simulink model "sm_car"  (R2025a)
settings: Solver=ode23t  StartTime=0.0  StopTime=400  MaxStep=0.4  RelTol=1e-3  AbsTol=1e-3  EnableMultiTasking=on
PreLoadFcn:
  | % Due to usability issue in Repeating Sequence block
  | warning('off','Simulink:Masking:Invalid');
  | 
  | % Eliminate unnecessary warnings in inactive variants
  | % Warnings generated only if you click through inactive variant
  | warning('off','MATLAB:nonExistentField');
  | warning('off','Simulink:Parameters:BlkParamUndefined');
PostLoadFcn:
  | set_param([bdroot '/Vehicle'],'popup_trailer','Off')
  | warning('off','sm:sli:setup:compile:LocalSolverNotSupported')
  | %sm_car_config_maneuver(bdroot,'WOT Braking');
  | sm_car_config_vehicle(bdroot,'false');
  | sm_car_config_logging(bdroot);
InitFcn:
  | sm_car_config_camera;
  | Vehicle = sm_car_vehcfg_checkConfig(Vehicle);
  | sm_car_check_tire_model(bdroot);
StartFcn:
  | tic;
StopFcn:
  | Elapsed_Sim_Time = toc;
  | % disp(['Elapsed Sim Time = ' num2str(Elapsed_Sim_Time)]);
undefined symbols (not defined in the file): Axle1D, AxleIn, Camera, Control, Driver, Free, Init, Maneuver, Pedal, RaceFix, RaceSpin, Scene, ShaftL1, ShaftL2, ShaftR1, ShaftR2, Soft, Stiff, Visual, X, xy_data_car_side, Y, Z
libraries: sm_lib x1546, nesl_utility x528, fl_lib x480, SimscapeFluids_lib x61, sdl_lib x49, simulink x29, ee_lib x7, simulink_extras x6, Linkage_Systems x4, Tire_1x2x x4, AntiRollBar_Systems x2, Linkage_Decoupled x2
(part 9 of 79)

== system sm_car/World/Scene/Skidpad/Circle Outer R ==
  Solid : sm_lib/Body Elements/Extruded Solid  ExtrusionType=General  PolygonNumSides=3  PolygonOuterRadius=1  PolygonOuterRadiusUnits=m  ExportEntireGeometry=off  ExtrusionCrossSection=xy_data_circ  ExtrusionCrossSectionUnits=m  ExportConvexHullGeometry=off  ExtrusionLength=circ_h  ExtrusionLengthUnits=m  InertiaType=CalculateFromGeometry  BasedOnType=Density  Density=1000  DensityUnits=kg/m^3  Mass=1  MassUnits=kg  CenterOfMass=[0 0 0]  CenterOfMassUnits=m  MomentsOfInertia=[1 1 1]  MomentsOfInertiaUnits=kg*m^2  ProductsOfInertia=[1 1 1]  ProductsOfInertiaUnits=kg*m^2  GraphicType=FromGeometry  MarkerShape=Sphere  MarkerSize=10  GraphicVisPropType=SimpleVisualProperties  GraphicDiffuseColor=[1.0 1.0 0.8]  GraphicOpacity=1.0  GraphicSpecularColor=[0.5 0.5 0.5 1.0]  GraphicAmbientColor=[0.15 0.15 0.15 1.0]  GraphicEmissiveColor=[0.0 0.0 0.0 1.0]  GraphicShininess=75  DoExposeReferenceFrame=on  SerializedFrames=<Frames/>
  W : PMIOPort  Side=Right
  connections:
  Solid/RConn1 -- W/RConn1

== system sm_car/World/Scene/Skidpad/Ground Plane ==
  Floor : sm_lib/Body Elements/Brick Solid  BrickDimensions=[gp_l, gp_w, gp_h]  BrickDimensionsUnits=m  ExportEntireGeometry=off  InertiaType=CalculateFromGeometry  BasedOnType=Density  Density=1000  DensityUnits=kg/m^3  Mass=1  MassUnits=kg  CenterOfMass=[0 0 0]  CenterOfMassUnits=m  MomentsOfInertia=[1 1 1]  MomentsOfInertiaUnits=kg*m^2  ProductsOfInertia=[0 0 0]  ProductsOfInertiaUnits=kg*m^2  GraphicType=FromGeometry  MarkerShape=Sphere  MarkerSize=10  GraphicVisPropType=SimpleVisualProperties  GraphicDiffuseColor=gp_clr  GraphicOpacity=gp_opc  GraphicSpecularColor=[0.5 0.5 0.5 1.0]  GraphicAmbientColor=[0.15 0.15 0.15 1.0]  GraphicEmissiveColor=[0.0 0.0 0.0 1.0]  GraphicShininess=75  DoExposeReferenceFrame=off  SerializedFrames=<Frames><Frame><Id>Frame1</Id><Value><Name>F</Name><Origin><Source>GeometricFeature</Source><FeatureName>+z surface</FeatureName></Origin><PrimaryAxis><DefinedDirection>+Z</DefinedDirection><Source>ReferenceFrame</Source><SourceDirection>+Z</SourceDirection><FeatureName></FeatureName></PrimaryAxis><SecondaryAxis><DefinedDirection>+X</DefinedDirection><Source>ReferenceFrame</Source><SourceDirection>+X</SourceDirection><FeatureName></FeatureName></SecondaryAxis></Value></Frame></Frames>
  W : PMIOPort  Side=Right
  connections:
  Floor/LConn1 -- W/RConn1

== system sm_car/Controller/Default/Damper Control/Damper Control A1/None ==
  mL : Inport
  mR : Inport  Port=2
  Inp : Inport  Port=3
  Ground : Ground
  Ground1 : Ground
  Terminator : Terminator
  Terminator1 : Terminator
  Terminator2 : Terminator
  L : Outport  VectorParamsAs1DForOutWhenUnconnected=off
  R : Outport  Port=2  VectorParamsAs1DForOutWhenUnconnected=off
  wires:
  Inp/1 -> Terminator2/1
  mR/1 -> Terminator1/1
  mL/1 -> Terminator/1
  Ground1/1 -> R/1  "R"
  Ground/1 -> L/1  "L"

== system sm_car/Controller/Default/Damper Control/Damper Control A2/None ==
  mL : Inport
  mR : Inport  Port=2
  Inp : Inport  Port=3
  Ground : Ground
  Ground1 : Ground
  Terminator : Terminator
  Terminator1 : Terminator
  Terminator2 : Terminator
  L : Outport  VectorParamsAs1DForOutWhenUnconnected=off
  R : Outport  Port=2  VectorParamsAs1DForOutWhenUnconnected=off
  wires:
  Inp/1 -> Terminator2/1
  mR/1 -> Terminator1/1
  mL/1 -> Terminator/1
  Ground1/1 -> R/1  "R"
  Ground/1 -> L/1  "L"

== system sm_car/Controller/Default/Spring Control/Spring Control A1/Hydropneumatic ==
  mL : Inport
  mR : Inport  Port=2
  Inp : Inport  Port=3
  Bus Creator : BusCreator  Inputs=5
  Constant : Constant  Value=0
  Constant1 : Constant  Value=0
  Gain : Gain
  Prop Damper : Constant  Value=0
  Soft Suspension : Constant  Value=soft_suspension
  Terminator : Terminator
  Terminator1 : Terminator
  Terminator2 : Terminator
  L : Outport  VectorParamsAs1DForOutWhenUnconnected=off
  R : Outport  Port=2  VectorParamsAs1DForOutWhenUnconnected=off
  wires:
  Bus Creator/1 -> R/1, L/1  "R"
  mL/1 -> Terminator/1
  mR/1 -> Terminator1/1
  Inp/1 -> Terminator2/1
  Constant1/1 -> Bus Creator/5  "RideHeightOut"
  Gain/1 -> Bus Creator/1  "GasSprStiff"
  Soft Suspension/1 -> Bus Creator/2, Gain/1  "GasSprSoft"
  Prop Damper/1 -> Bus Creator/3  "Damper"
  Constant/1 -> Bus Creator/4  "RideHeightIn"

== system sm_car/Controller/Default/Spring Control/Spring Control A1/None ==
  mL : Inport
  mR : Inport  Port=2
  Inp : Inport  Port=3
  Ground : Ground
  Ground1 : Ground
  Terminator1 : Terminator
  Terminator2 : Terminator
  Terminator3 : Terminator
  L : Outport  VectorParamsAs1DForOutWhenUnconnected=off
  R : Outport  Port=2  VectorParamsAs1DForOutWhenUnconnected=off
  wires:
  Inp/1 -> Terminator3/1
  Ground/1 -> L/1  "L"
  Ground1/1 -> R/1  "R"
  mL/1 -> Terminator1/1
  mR/1 -> Terminator2/1

== system sm_car/Controller/Default/Spring Control/Spring Control A2/Hydropneumatic ==
  mL : Inport
  mR : Inport  Port=2
  Inp : Inport  Port=3
  Bus Creator : BusCreator  Inputs=5
  Constant : Constant  Value=0
  Constant1 : Constant  Value=0
  Gain : Gain
  Prop Damper : Constant  Value=0
  Soft Suspension : Constant  Value=soft_suspension
  Terminator : Terminator
  Terminator1 : Terminator
  Terminator2 : Terminator
  L : Outport  VectorParamsAs1DForOutWhenUnconnected=off
  R : Outport  Port=2  VectorParamsAs1DForOutWhenUnconnected=off
  wires:
  Bus Creator/1 -> R/1, L/1  "R"
  mL/1 -> Terminator/1
  mR/1 -> Terminator1/1
  Inp/1 -> Terminator2/1
  Constant1/1 -> Bus Creator/5  "RideHeightOut"
  Gain/1 -> Bus Creator/1  "GasSprStiff"
  Soft Suspension/1 -> Bus Creator/2, Gain/1  "GasSprSoft"
  Prop Damper/1 -> Bus Creator/3  "Damper"
  Constant/1 -> Bus Creator/4  "RideHeightIn"

== system sm_car/Controller/Default/Spring Control/Spring Control A2/None ==
  mL : Inport
  mR : Inport  Port=2
  Inp : Inport  Port=3
  Ground : Ground
  Ground1 : Ground
  Terminator1 : Terminator
  Terminator2 : Terminator
  Terminator3 : Terminator
  L : Outport  VectorParamsAs1DForOutWhenUnconnected=off
  R : Outport  Port=2  VectorParamsAs1DForOutWhenUnconnected=off
  wires:
  Inp/1 -> Terminator3/1
  Ground/1 -> L/1  "L"
  Ground1/1 -> R/1  "R"
  mL/1 -> Terminator1/1
  mR/1 -> Terminator2/1

== system sm_car/Controller/TrqVec 4Motor/Brake Control/ABS/Calculate Slip ==
  WhlSpd : Inport
  VehSpdEst : Inport  Port=2
  Abs : Abs  ZeroCross=off  SaturateOnIntegerOverflow=off
  Bus Creator : BusCreator  Inputs=4
  Bus Selector1 : BusSelector  OutputSignals=L1.v,R1.v,L2.v,R2.v
  Constant : Constant
  Demux : Demux
  Fcn{,1..3} (4 alike) : Fcn  Expr=abs(u(1)*u(2)-u(3))/u(3)
  Mux{,1..3} (4 alike) : Mux  Inputs=3
  Mux4 : Mux
  Mux5 : Mux
  Product : Product
  Saturation : Saturate  UpperLimit=inf  LowerLimit=eps  ZeroCross=off
  Saturation1 : Saturate  UpperLimit=1  LowerLimit=0
  Sign : Signum  ZeroCross=off
  Wheel Speeds and Slip : Scope  NumInputPorts=2
      settings: ActiveDisplayYMinimum=-11.64241  ActiveDisplayYMaximum=114.01232  DataLoggingVariableName=ScopeData2
  Slip : Outport  VectorParamsAs1DForOutWhenUnconnected=off
  wires:
  WhlSpd/1 -> Bus Selector1/1
  Bus Selector1/2 -> Mux4/2, Mux1/2  "<v>"
  Bus Selector1/4 -> Mux4/4, Mux3/2  "<v>"
  Bus Selector1/1 -> Mux4/1, Mux/2  "<v>"
  Bus Selector1/3 -> Mux4/3, Mux2/2  "<v>"
  Constant/1 -> Mux/1, Mux1/1, Mux3/1, Mux2/1
  VehSpdEst/1 -> Sign/1, Abs/1
  Demux/1 -> Bus Creator/1  "L1"
  Demux/2 -> Bus Creator/2  "R1"
  Demux/3 -> Bus Creator/3  "L2"
  Demux/4 -> Bus Creator/4  "R2"
  Bus Creator/1 -> Wheel Speeds and Slip/2, Slip/1  "Slip"
  Product/1 -> Mux3/3, Mux2/3, Mux1/3, Mux/3
  Abs/1 -> Saturation/1
  Saturation/1 -> Product/1
  Sign/1 -> Product/2
  Mux/1 -> Fcn/1
  Mux1/1 -> Fcn1/1
  Mux2/1 -> Fcn2/1
  Mux3/1 -> Fcn3/1
  Mux4/1 -> Wheel Speeds and Slip/1  "Wheel Speeds"
  Mux5/1 -> Saturation1/1
  Saturation1/1 -> Demux/1
  Fcn/1 -> Mux5/1  "L1"
  Fcn1/1 -> Mux5/2  "R1"
  Fcn2/1 -> Mux5/3  "L2"
  Fcn3/1 -> Mux5/4  "R2"

== system sm_car/Controller/TrqVec 4Motor/Brake Control/ABS/Sensor ==
  Body : Inport
  WhlSpd : Inport  Port=2
  Bus Creator{,3..5} (4 alike) : BusCreator  Inputs=1
  Bus Creator6 : BusCreator  Inputs=5
  Bus Selector : BusSelector  OutputSignals=vx,vy  OutputAsBus=on
  Bus Selector4 : BusSelector  OutputSignals=WhlL1.n,WhlR1.n,WhlL2.n,WhlR2.n,WhlL2.qxyz
  Gain : Gain  Gain=3.6*abs_tire_radiusF
  Gain1 : Gain  Gain=3.6*abs_tire_radiusF
  Gain2 : Gain  Gain=3.6*abs_tire_radiusR
  Gain3 : Gain  Gain=3.6*abs_tire_radiusR
  Gain4 : Gain  Gain=3.6
  Terminator1 : Terminator  Commented=on
  Vel in xy plane : Fcn  Expr=sqrt(u(1)^2+u(2)^2)
  missing tooth : Subsystem  Commented=on
  GroundSpd : Outport  VectorParamsAs1DForOutWhenUnconnected=off
  wires:
  Gain1/1 -> Bus Creator3/1  "v"
  missing tooth/1(Out1) -> Terminator1/1  "v"
  Gain2/1 -> Bus Creator4/1  "v"
  Bus Selector4/5 -> missing tooth/2(<qxyz>)  "<qxyz>"
  Bus Creator5/1 -> Bus Creator6/5  "R2"
  Gain3/1 -> Bus Creator5/1  "v"
  Bus Creator/1 -> Bus Creator6/2  "L1"
  Bus Selector4/2 -> Gain1/1  "<n>"
  Bus Creator4/1 -> Bus Creator6/4  "L2"
  Bus Selector4/3 -> Gain2/1, missing tooth/1(<omega>)  "<n>"
  Gain/1 -> Bus Creator/1  "v"
  Body/1 -> Bus Selector/1
  Bus Creator3/1 -> Bus Creator6/3  "R1"
  Gain4/1 -> Bus Creator6/1  "v"
  Bus Selector4/1 -> Gain/1  "<n>"
  Bus Selector4/4 -> Gain3/1  "<n>"
  WhlSpd/1 -> Bus Selector4/1
  Bus Creator6/1 -> GroundSpd/1
  Vel in xy plane/1 -> Gain4/1  "speed"
  Bus Selector/1 -> Vel in xy plane/1

== system sm_car/Controller/TrqVec 4Motor/Brake Control/ABS/Valve Control L1 ==
  Slip : Inport
  vSpdEst : Inport  Port=2
  Categorize Surface : Subsystem
  Code to Valves : Subsystem
  Demux : Demux  Outputs=2
  Logic : Stateflow chart  TreatAsAtomicUnit=on
  Mux : Mux  Inputs=2
  Product : Product
  Subsystem : Subsystem
  Subsystem1 : Subsystem
  Valve : Outport  VectorParamsAs1DForOutWhenUnconnected=off
  wires:
  Logic/1(Mod_State) -> Categorize Surface/1(Mod State), Code to Valves/1(C)
  Logic/2(Mod_Dur) -> Product/2
  Slip/1 -> Logic/1(Slip)
  Code to Valves/1(V) -> Product/1
  vSpdEst/1 -> Logic/2(vSpdEst)
  Product/1 -> Demux/1
  Demux/1 -> Subsystem/1(OnT)
  Demux/2 -> Subsystem1/1(OnT)
  Mux/1 -> Valve/1
  Subsystem/1(vSig) -> Mux/1, Categorize Surface/2(Apply Valve)
  Subsystem1/1(vSig) -> Mux/2

== system sm_car/Controller/TrqVec 4Motor/Brake Control/ABS/Valve Control L2 ==
  Slip : Inport
  vSpdEst : Inport  Port=2
  Categorize Surface : Subsystem
  Code to Valves : Subsystem
  Demux : Demux  Outputs=2
  Logic : Stateflow chart  TreatAsAtomicUnit=on
  Mux : Mux  Inputs=2
  Product : Product
  Subsystem : Subsystem
  Subsystem1 : Subsystem
  Valve : Outport  VectorParamsAs1DForOutWhenUnconnected=off
  wires:
  Logic/1(Mod_State) -> Categorize Surface/1(Mod State), Code to Valves/1(C)
  Logic/2(Mod_Dur) -> Product/2
  Slip/1 -> Logic/1(Slip)
  Code to Valves/1(V) -> Product/1
  vSpdEst/1 -> Logic/2(vSpdEst)
  Product/1 -> Demux/1
  Demux/1 -> Subsystem/1(OnT)
  Demux/2 -> Subsystem1/1(OnT)
  Mux/1 -> Valve/1
  Subsystem/1(vSig) -> Mux/1, Categorize Surface/2(Apply Valve)
  Subsystem1/1(vSig) -> Mux/2

== system sm_car/Controller/TrqVec 4Motor/Brake Control/ABS/Valve Control R1 ==
  Slip : Inport
  vSpdEst : Inport  Port=2
  Categorize Surface : Subsystem
  Code to Valves : Subsystem
  Demux : Demux  Outputs=2
  Logic : Stateflow chart  TreatAsAtomicUnit=on
  Mux : Mux  Inputs=2
  Product : Product
  Subsystem : Subsystem
  Subsystem1 : Subsystem
  Valve : Outport  VectorParamsAs1DForOutWhenUnconnected=off
  wires:
  Logic/1(Mod_State) -> Categorize Surface/1(Mod State), Code to Valves/1(C)
  Logic/2(Mod_Dur) -> Product/2
  Slip/1 -> Logic/1(Slip)
  Code to Valves/1(V) -> Product/1
  vSpdEst/1 -> Logic/2(vSpdEst)
  Product/1 -> Demux/1
  Demux/1 -> Subsystem/1(OnT)
  Demux/2 -> Subsystem1/1(OnT)
  Mux/1 -> Valve/1
  Subsystem/1(vSig) -> Mux/1, Categorize Surface/2(Apply Valve)
  Subsystem1/1(vSig) -> Mux/2

== system sm_car/Controller/TrqVec 4Motor/Brake Control/ABS/Valve Control R2 ==
  Slip : Inport
  vSpdEst : Inport  Port=2
  Categorize Surface : Subsystem
  Code to Valves : Subsystem
  Demux : Demux  Outputs=2
  Logic : Stateflow chart  TreatAsAtomicUnit=on
  Mux : Mux  Inputs=2
  Product : Product
  Subsystem : Subsystem
  Subsystem1 : Subsystem
  Valve : Outport  VectorParamsAs1DForOutWhenUnconnected=off
  wires:
  Logic/1(Mod_State) -> Categorize Surface/1(Mod State), Code to Valves/1(C)
  Logic/2(Mod_Dur) -> Product/2
  Slip/1 -> Logic/1(Slip)
  Code to Valves/1(V) -> Product/1
  vSpdEst/1 -> Logic/2(vSpdEst)
  Product/1 -> Demux/1
  Demux/1 -> Subsystem/1(OnT)
  Demux/2 -> Subsystem1/1(OnT)
  Mux/1 -> Valve/1
  Subsystem/1(vSig) -> Mux/1, Categorize Surface/2(Apply Valve)
  Subsystem1/1(vSig) -> Mux/2

== system sm_car/Controller/TrqVec 4Motor/Brake Control/ABS/Vehicle Speed ==
  Sensors : Inport
  Bus Selector : BusSelector  OutputSignals=v
  vSpdEst : Outport  VectorParamsAs1DForOutWhenUnconnected=off
  wires:
  Sensors/1 -> Bus Selector/1
  Bus Selector/1 -> vSpdEst/1  "<v>"

== system sm_car/Controller/TrqVec 4Motor/Damper Control/Damper Control A1/Coefficient ==
  mL : Inport
  mR : Inport  Port=2
  Inp : Inport  Port=3
  Bus Selector : BusSelector  OutputSignals=vDamper
  Bus Selector1 : BusSelector  OutputSignals=vDamper
  Demux : Demux  Outputs=2
  Filter : Subsystem  mask(First-order lag supporting vector signals){b=b_A1, x_initial=[0 0]}
      mask prompts: b "Filter time constant"; x_initial "Initial output"
      mask help: Models a lag of the form 1/(b*s+1) where s is the Laplace operator.
  Lookup Table Coeff : Lookup_n-D  BreakpointsForDimension1=brkPts_dim1_A1  BreakpointsForDimension2=brkPts_dim2_A1  Table=Table_A1  InternalRulePriority=Speed  RndMeth=Simplest
      settings: InputPortMap=u0,u1
  Mux1 : Mux  Inputs=2
  L : Outport  VectorParamsAs1DForOutWhenUnconnected=off
  R : Outport  Port=2  VectorParamsAs1DForOutWhenUnconnected=off
  wires:
  Bus Selector1/1 -> Mux1/2  "<vDamper>"
  mR/1 -> Bus Selector1/1
  mL/1 -> Bus Selector/1
  Filter/1(Out) -> Lookup Table Coeff/1  "vDamper"
  Bus Selector/1 -> Mux1/1  "<vDamper>"
  Mux1/1 -> Filter/1(In)
  Demux/1 -> L/1  "L"
  Demux/2 -> R/1  "R"
  Inp/1 -> Lookup Table Coeff/2
  Lookup Table Coeff/1 -> Demux/1  "dDamper"

== system sm_car/Controller/TrqVec 4Motor/Damper Control/Damper Control A1/Force ==
  mL : Inport
  mR : Inport  Port=2
  Inp : Inport  Port=3
  Bus Selector : BusSelector  OutputSignals=vDamper
  Bus Selector1 : BusSelector  OutputSignals=vDamper
  Demux : Demux  Outputs=2
  Filter : Subsystem  mask(First-order lag supporting vector signals){b=b_A1, x_initial=[0 0]}
      mask prompts: b "Filter time constant"; x_initial "Initial output"
      mask help: Models a lag of the form 1/(b*s+1) where s is the Laplace operator.
  Lookup Table A1 : Lookup_n-D  BreakpointsForDimension1=brkPts_dim1_A1  BreakpointsForDimension2=brkPts_dim2_A1  Table=Table_A1  InternalRulePriority=Speed  RndMeth=Simplest
      settings: InputPortMap=u0,u1
  Mux1 : Mux  Inputs=2
  L : Outport  VectorParamsAs1DForOutWhenUnconnected=off
  R : Outport  Port=2  VectorParamsAs1DForOutWhenUnconnected=off
  wires:
  Bus Selector1/1 -> Mux1/2  "<vDamper>"
  mR/1 -> Bus Selector1/1
  mL/1 -> Bus Selector/1
  Filter/1(Out) -> Lookup Table A1/1  "vDamper"
  Bus Selector/1 -> Mux1/1  "<vDamper>"
  Mux1/1 -> Filter/1(In)
  Demux/1 -> L/1  "L"
  Demux/2 -> R/1  "R"
  Inp/1 -> Lookup Table A1/2
  Lookup Table A1/1 -> Demux/1  "fDamper"

== system sm_car/Controller/TrqVec 4Motor/Damper Control/Damper Control A1/None ==
  mL : Inport
  mR : Inport  Port=2
  Inp : Inport  Port=3
  Ground : Ground
  Ground1 : Ground
  Terminator : Terminator
  Terminator1 : Terminator
  Terminator2 : Terminator
  L : Outport  VectorParamsAs1DForOutWhenUnconnected=off
  R : Outport  Port=2  VectorParamsAs1DForOutWhenUnconnected=off
  wires:
  Inp/1 -> Terminator2/1
  mR/1 -> Terminator1/1
  mL/1 -> Terminator/1
  Ground1/1 -> R/1  "R"
  Ground/1 -> L/1  "L"

== system sm_car/Controller/TrqVec 4Motor/Damper Control/Damper Control A2/Coefficient ==
  mL : Inport
  mR : Inport  Port=2
  Inp : Inport  Port=3
  Bus Selector : BusSelector  OutputSignals=vDamper
  Bus Selector1 : BusSelector  OutputSignals=vDamper
  Demux : Demux  Outputs=2
  Filter : Subsystem  mask(First-order lag supporting vector signals){b=b_A1, x_initial=[0 0]}
      mask prompts: b "Filter time constant"; x_initial "Initial output"
      mask help: Models a lag of the form 1/(b*s+1) where s is the Laplace operator.
  Lookup Table Coeff : Lookup_n-D  BreakpointsForDimension1=brkPts_dim1_A1  BreakpointsForDimension2=brkPts_dim2_A1  Table=Table_A1  InternalRulePriority=Speed  RndMeth=Simplest
      settings: InputPortMap=u0,u1
  Mux1 : Mux  Inputs=2
  L : Outport  VectorParamsAs1DForOutWhenUnconnected=off
  R : Outport  Port=2  VectorParamsAs1DForOutWhenUnconnected=off
  wires:
  Bus Selector1/1 -> Mux1/2  "<vDamper>"
  mR/1 -> Bus Selector1/1
  mL/1 -> Bus Selector/1
  Filter/1(Out) -> Lookup Table Coeff/1  "vDamper"
  Bus Selector/1 -> Mux1/1  "<vDamper>"
  Mux1/1 -> Filter/1(In)
  Demux/1 -> L/1  "L"
  Demux/2 -> R/1  "R"
  Inp/1 -> Lookup Table Coeff/2
  Lookup Table Coeff/1 -> Demux/1  "dDamper"

== system sm_car/Controller/TrqVec 4Motor/Damper Control/Damper Control A2/Force ==
  mL : Inport
  mR : Inport  Port=2
  Inp : Inport  Port=3
  Bus Selector : BusSelector  OutputSignals=vDamper
  Bus Selector1 : BusSelector  OutputSignals=vDamper
  Demux : Demux  Outputs=2
  Filter : Subsystem  mask(First-order lag supporting vector signals){b=b_A1, x_initial=[0 0]}
      mask prompts: b "Filter time constant"; x_initial "Initial output"
      mask help: Models a lag of the form 1/(b*s+1) where s is the Laplace operator.
  Lookup Table A1 : Lookup_n-D  BreakpointsForDimension1=brkPts_dim1_A1  BreakpointsForDimension2=brkPts_dim2_A1  Table=Table_A1  InternalRulePriority=Speed  RndMeth=Simplest
      settings: InputPortMap=u0,u1
  Mux1 : Mux  Inputs=2
  L : Outport  VectorParamsAs1DForOutWhenUnconnected=off
  R : Outport  Port=2  VectorParamsAs1DForOutWhenUnconnected=off
  wires:
  Bus Selector1/1 -> Mux1/2  "<vDamper>"
  mR/1 -> Bus Selector1/1
  mL/1 -> Bus Selector/1
  Filter/1(Out) -> Lookup Table A1/1  "vDamper"
  Bus Selector/1 -> Mux1/1  "<vDamper>"
  Mux1/1 -> Filter/1(In)
  Demux/1 -> L/1  "L"
  Demux/2 -> R/1  "R"
  Inp/1 -> Lookup Table A1/2
  Lookup Table A1/1 -> Demux/1  "fDamper"

== system sm_car/Controller/TrqVec 4Motor/Damper Control/Damper Control A2/None ==
  mL : Inport
  mR : Inport  Port=2
  Inp : Inport  Port=3
  Ground : Ground
  Ground1 : Ground
  Terminator : Terminator
  Terminator1 : Terminator
  Terminator2 : Terminator
  L : Outport  VectorParamsAs1DForOutWhenUnconnected=off
  R : Outport  Port=2  VectorParamsAs1DForOutWhenUnconnected=off
  wires:
  Inp/1 -> Terminator2/1
  mR/1 -> Terminator1/1
  mL/1 -> Terminator/1
  Ground1/1 -> R/1  "R"
  Ground/1 -> L/1  "L"

== system sm_car/Controller/TrqVec 4Motor/Power_TqVec/Torque Vectoring/Accel Torque Request ==
  note: Assumes both rear motors have same torque speed curve
  MotSpdL2 : Inport
  MotSpdR2 : Inport  Port=2
  MaxMotTrqVsSpdA1 : Lookup_n-D  NumberOfTableDimensions=1  BreakpointsForDimension1=Control.MotorL2.TorqueSpd.w.Value  Table=Control.MotorL2.TorqueSpd.trq.Value  ExtrapMethod=Clip  UseLastTableValue=on  InternalRulePriority=Speed  OutDataTypeStr=Inherit: Inherit from 'Table data'  RndMeth=Simplest
  Terminator : Terminator
  rads_to_rpm : Gain  Gain=30/pi
  rads_to_rpm1 : Gain  Gain=30/pi
  TrqMax : Outport  VectorParamsAs1DForOutWhenUnconnected=off
  wires:
  rads_to_rpm1/1 -> Terminator/1
  MotSpdR2/1 -> rads_to_rpm1/1
  MaxMotTrqVsSpdA1/1 -> TrqMax/1
  MotSpdL2/1 -> rads_to_rpm/1
  rads_to_rpm/1 -> MaxMotTrqVsSpdA1/1

== system sm_car/Controller/TrqVec 4Motor/Power_TqVec/Torque Vectoring/Enable ==
  note: Ramp up amount of torque vectoring over a range.
  note: Steer angle threshold to enable torque vectoring
  vx : Inport
  aSteerWheel : Inport  Port=2
  Abs : Abs  ZeroCross=off  SaturateOnIntegerOverflow=off
  Data Type Conversion : DataTypeConversion  OutDataTypeStr=double  SaturateOnIntegerOverflow=off  RndMeth=Floor
  Divide : Product  Inputs=*/
  Enable vx : simulink/Logic and Bit Operations/Compare To Constant  relop=>  const=vx_enable  OutDataTypeStr=boolean  ZeroCross=off
  Gain : Gain  Gain=0.25
  Product : Product
  Saturation : Saturate  UpperLimit=1  LowerLimit=0  ZeroCross=off
  Subtract : Sum  Inputs=+-
  const : Constant  Value=aSteerWheel_enable
  Enable : Outport  VectorParamsAs1DForOutWhenUnconnected=off
  wires:
  Gain/1 -> Divide/1
  Product/1 -> Enable/1
  Divide/1 -> Saturation/1
  Subtract/1 -> Gain/1
  Abs/1 -> Subtract/1
  Saturation/1 -> Product/2
  Data Type Conversion/1 -> Product/1
  Enable vx/1 -> Data Type Conversion/1
  const/1 -> Subtract/2, Divide/2
  aSteerWheel/1 -> Abs/1
  vx/1 -> Enable vx/1

== system sm_car/Controller/TrqVec 4Motor/Power_TqVec/Torque Vectoring/Vehicle Slip Angle Error ==
  vx : Inport
  aSteerWheel : Inport  Port=2
  nYaw : Inport  Port=3
  Add1 : Sum  Inputs=-+
  Distance Yaw Ctr Front Axle : Constant  Value=Vehicle.Chassis.Body.sAxle2.Value(1)/(-2)
  Divide3 : Product  Inputs=*/
  Multiply2 : Product
  Mux : Mux  Inputs=2
  Scope : Scope  NumInputPorts=2
      settings: ActiveDisplayYMinimum=-0.04829  ActiveDisplayYMaximum=0.00545
  Steering Wheel to Driving Wheel : Gain  Gain=aStr_to_aWhl
  Error : Outport  VectorParamsAs1DForOutWhenUnconnected=off
  wires:
  Mux/1 -> Scope/1
  Multiply2/1 -> Divide3/1
  Steering Wheel to Driving Wheel/1 -> Mux/2, Add1/2  "Wheel Angle"
  Distance Yaw Ctr Front Axle/1 -> Multiply2/1
  aSteerWheel/1 -> Steering Wheel to Driving Wheel/1
  nYaw/1 -> Multiply2/2
  Add1/1 -> Scope/2, Error/1  "Error"
  vx/1 -> Divide3/2
  Divide3/1 -> Add1/1, Mux/1  "Vehicle Slip Angle"

== system sm_car/Controller/TrqVec 4Motor/Spring Control/Spring Control A1/Hydropneumatic ==
  mL : Inport
  mR : Inport  Port=2
  Inp : Inport  Port=3
  Bus Creator : BusCreator  Inputs=5
  Constant : Constant  Value=0
  Constant1 : Constant  Value=0
  Gain : Gain
  Prop Damper : Constant  Value=0
  Soft Suspension : Constant  Value=soft_suspension
  Terminator : Terminator
  Terminator1 : Terminator
  Terminator2 : Terminator
  L : Outport  VectorParamsAs1DForOutWhenUnconnected=off
  R : Outport  Port=2  VectorParamsAs1DForOutWhenUnconnected=off
  wires:
  Bus Creator/1 -> R/1, L/1  "R"
  mL/1 -> Terminator/1
  mR/1 -> Terminator1/1
  Inp/1 -> Terminator2/1
  Constant1/1 -> Bus Creator/5  "RideHeightOut"
  Gain/1 -> Bus Creator/1  "GasSprStiff"
  Soft Suspension/1 -> Bus Creator/2, Gain/1  "GasSprSoft"
  Prop Damper/1 -> Bus Creator/3  "Damper"
  Constant/1 -> Bus Creator/4  "RideHeightIn"

== system sm_car/Controller/TrqVec 4Motor/Spring Control/Spring Control A1/None ==
  mL : Inport
  mR : Inport  Port=2
  Inp : Inport  Port=3
  Ground : Ground
  Ground1 : Ground
  Terminator1 : Terminator
  Terminator2 : Terminator
  Terminator3 : Terminator
  L : Outport  VectorParamsAs1DForOutWhenUnconnected=off
  R : Outport  Port=2  VectorParamsAs1DForOutWhenUnconnected=off
  wires:
  Inp/1 -> Terminator3/1
  Ground/1 -> L/1  "L"
  Ground1/1 -> R/1  "R"
  mL/1 -> Terminator1/1
  mR/1 -> Terminator2/1

== system sm_car/Controller/TrqVec 4Motor/Spring Control/Spring Control A2/Hydropneumatic ==
  mL : Inport
  mR : Inport  Port=2
  Inp : Inport  Port=3
  Bus Creator : BusCreator  Inputs=5
  Constant : Constant  Value=0
  Constant1 : Constant  Value=0
  Gain : Gain
  Prop Damper : Constant  Value=0
  Soft Suspension : Constant  Value=soft_suspension
  Terminator : Terminator
  Terminator1 : Terminator
  Terminator2 : Terminator
  L : Outport  VectorParamsAs1DForOutWhenUnconnected=off
  R : Outport  Port=2  VectorParamsAs1DForOutWhenUnconnected=off
  wires:
  Bus Creator/1 -> R/1, L/1  "R"
  mL/1 -> Terminator/1
  mR/1 -> Terminator1/1
  Inp/1 -> Terminator2/1
  Constant1/1 -> Bus Creator/5  "RideHeightOut"
  Gain/1 -> Bus Creator/1  "GasSprStiff"
  Soft Suspension/1 -> Bus Creator/2, Gain/1  "GasSprSoft"
  Prop Damper/1 -> Bus Creator/3  "Damper"
  Constant/1 -> Bus Creator/4  "RideHeightIn"

== system sm_car/Controller/TrqVec 4Motor/Spring Control/Spring Control A2/None ==
  mL : Inport
  mR : Inport  Port=2
  Inp : Inport  Port=3
  Ground : Ground
  Ground1 : Ground
  Terminator1 : Terminator
  Terminator2 : Terminator
  Terminator3 : Terminator
  L : Outport  VectorParamsAs1DForOutWhenUnconnected=off
  R : Outport  Port=2  VectorParamsAs1DForOutWhenUnconnected=off
  wires:
  Inp/1 -> Terminator3/1
  Ground/1 -> L/1  "L"
  Ground1/1 -> R/1  "R"
  mL/1 -> Terminator1/1
  mR/1 -> Terminator2/1

== system sm_car/Driver/Closed Loop/Driver/Lateral Driver/Pure Pursuit ==
  referencePose : Inport
  Distance : Inport  Port=2
  currentPose : Inport  Port=3
  v_x : Inport  Port=4
  Preview : Inport  Port=5
  Direction : Inport  Port=6
  Bus Selector : BusSelector  OutputSignals=pp_preview_x_pts,pp_preview_dist_pts,pp_preview_y_pts,pp_preview_yaw_pts
  Constant : Constant  Value=MAX_STEERING_ANGLE_DEG
  Constant1 : Constant  Value=L_AXLE_DIST
  Constant5 : Constant  Value=LOOKAHEAD_GAIN_KPP
  Constant6 : Constant  Value=MAX_LOOKAHEAD_DIST
  Constant7 : Constant  Value=MIN_LOOKAHEAD_DIST
  Constant8 : Constant  Value=HEADING_WEIGHT_KH
  MATLAB Function1 : MATLAB Function  TreatAsAtomicUnit=on
  Terminator : Terminator
  steeringAngle : Outport
  wires:
  referencePose/1 -> Terminator/1
  v_x/1 -> MATLAB Function1/7(v_x)
  currentPose/1 -> MATLAB Function1/6(currentPose)
  Direction/1 -> MATLAB Function1/8(direction)
  Constant/1 -> MATLAB Function1/10(MAX_STEERING_ANGLE_DEG)
  Constant1/1 -> MATLAB Function1/9(L_AXLE_DIST)
  MATLAB Function1/1(steeringAngle) -> steeringAngle/1
  Constant5/1 -> MATLAB Function1/11(LOOKAHEAD_GAIN_KPP)
  Constant6/1 -> MATLAB Function1/13(MAX_LOOKAHEAD_DIST)
  Constant7/1 -> MATLAB Function1/12(MIN_LOOKAHEAD_DIST)
  Preview/1 -> Bus Selector/1
  Distance/1 -> MATLAB Function1/5(ad_vehicle)
  Bus Selector/1 -> MATLAB Function1/1(pp_preview_x_pts)  "<pp_preview_x_pts>"
  Bus Selector/2 -> MATLAB Function1/2(pp_preview_dist_pts)  "<pp_preview_dist_pts>"
  Bus Selector/3 -> MATLAB Function1/3(pp_preview_y_pts)  "<pp_preview_y_pts>"
  Bus Selector/4 -> MATLAB Function1/4(pp_preview_yaw_pts)  "<pp_preview_yaw_pts>"
  Constant8/1 -> MATLAB Function1/14(HEADING_WEIGHT_KH)

== system sm_car/Driver/Closed Loop/Driver/Lateral Driver/Stanley ==
  referencePose : Inport
  Distance : Inport  Port=2
  currentPose : Inport  Port=3
  v_x : Inport  Port=4
  Preview : Inport  Port=5
  Direction : Inport  Port=6
  Constant : Constant  Value=MAX_STEERING_ANGLE_DEG
  Constant1 : Constant  Value=L_AXLE_DIST
  Constant2 : Constant  Value=K_cte_forward
  Constant3 : Constant  Value=K_cte_reverse
  Stanley Driver : MATLAB Function  TreatAsAtomicUnit=on  mask(Lateral Driver (Stanley Driver)){}
      mask help:
      | Implements Stanley method for lateral control.
      | Supports forward and reverse driving.
      | Based on Hoffmann et al. (2007), "Autonomous Automobile Trajectory Tracking for Off-Road Driving"
  Terminator : Terminator
  Terminator1 : Terminator
  steeringAngle : Outport
  wires:
  Distance/1 -> Terminator1/1
  Preview/1 -> Terminator/1
  Stanley Driver/1(steeringAngle) -> steeringAngle/1
  Constant3/1 -> Stanley Driver/8(K_cte_reverse)
  Constant2/1 -> Stanley Driver/7(K_cte_forward)
  Constant1/1 -> Stanley Driver/5(L_AXLE_DIST)
  Constant/1 -> Stanley Driver/6(MAX_STEERING_ANGLE_DEG)
  referencePose/1 -> Stanley Driver/1(referencePose)
  Direction/1 -> Stanley Driver/4(direction)
  currentPose/1 -> Stanley Driver/2(currentPose)
  v_x/1 -> Stanley Driver/3(v_x)

== system sm_car/Driver/Closed Loop/Driver/Longitudinal Driver/Braking ==
  Constant17 : Constant  Value=gGravity
  Constant18 : Constant  Value=ROAD_FRICTION_COEFF
  Constant19 : Constant  Value=mVehicle
  Product1 : Product  Inputs=3
  myu*g*m : Outport
  wires:
  Constant19/1 -> Product1/3
  Constant18/1 -> Product1/1
  Product1/1 -> myu*g*m/1  "myu*g*m"
  Constant17/1 -> Product1/2

== system sm_car/Driver/Closed Loop/Driver/Longitudinal Driver/Drag ==
  Constant13 : Constant  Value=rho_air
  Constant15 : Constant  Value=0.5
  Constant16 : Constant  Value=ARef
  Constant5 : Constant  Value=Cdrag
  Product : Product  Inputs=4
  0.5*Cd*rho*A : Outport
  wires:
  Product/1 -> 0.5*Cd*rho*A/1  "0.5*Cd*rho*A"
  Constant16/1 -> Product/4
  Constant5/1 -> Product/2
  Constant13/1 -> Product/3
  Constant15/1 -> Product/1

== system sm_car/Driver/Closed Loop/Maneuver/Count Lap/Triggered Subsystem ==
  Up Down : Inport
  Trigger : TriggerPort  VariantControl=Variant  ZeroCross=off
  Memory : Memory  InheritSampleTime=on
  Sum : Sum  Inputs=|++
  Num Laps : Outport  VectorParamsAs1DForOutWhenUnconnected=off
  wires:
  Memory/1 -> Sum/1
  Sum/1 -> Memory/1, Num Laps/1
  Up Down/1 -> Sum/2

== system sm_car/Driver/Closed Loop/Maneuver/PoseTarget Visual/Pace Car ==
  Left Face : sm_lib/Body Elements/Extruded Solid  ExtrusionType=General  PolygonNumSides=3  PolygonOuterRadius=1  PolygonOuterRadiusUnits=m  ExportEntireGeometry=off  ExtrusionCrossSection=xy_data_car_side  ExtrusionCrossSectionUnits=m  ExportConvexHullGeometry=off  ExtrusionLength=thk_side  ExtrusionLengthUnits=m  InertiaType=PointMass  BasedOnType=Density  Density=1000  DensityUnits=kg/m^3  Mass=0  MassUnits=kg  CenterOfMass=[0 0 0]  CenterOfMassUnits=m  MomentsOfInertia=[1 1 1]  MomentsOfInertiaUnits=kg*m^2  ProductsOfInertia=[0 0 0]  ProductsOfInertiaUnits=kg*m^2  GraphicType=FromGeometry  MarkerShape=Sphere  MarkerSize=10  GraphicVisPropType=SimpleVisualProperties  GraphicDiffuseColor=clr_body_geo_left  GraphicOpacity=opc_body_geo_left  GraphicSpecularColor=[0.5 0.5 0.5 1.0]  GraphicAmbientColor=[0.15 0.15 0.15 1.0]  GraphicEmissiveColor=[0.0 0.0 0.0 1.0]  GraphicShininess=75  DoExposeReferenceFrame=on  SerializedFrames=<Frames/>
  Ornament Front : sm_lib/Body Elements/Extruded Solid  ExtrusionType=General  PolygonNumSides=3  PolygonOuterRadius=1  PolygonOuterRadiusUnits=m  ExportEntireGeometry=off  ExtrusionCrossSection=extr_data_emblem_f  ExtrusionCrossSectionUnits=m  ExportConvexHullGeometry=off  ExtrusionLength=0.01  ExtrusionLengthUnits=m  InertiaType=CalculateFromGeometry  BasedOnType=Density  Density=1000  DensityUnits=kg/m^3  Mass=1  MassUnits=kg  CenterOfMass=[0 0 0]  CenterOfMassUnits=m  MomentsOfInertia=[1 1 1]  MomentsOfInertiaUnits=kg*m^2  ProductsOfInertia=[0 0 0]  ProductsOfInertiaUnits=kg*m^2  GraphicType=FromGeometry  MarkerShape=Sphere  MarkerSize=10  GraphicVisPropType=AdvancedVisualProperties  GraphicDiffuseColor=clr_emblem_f  GraphicOpacity=opc_emblem_f  GraphicSpecularColor=[0.5 0.5 0.5 1.0]  GraphicAmbientColor=[0.15 0.15 0.15 1.0]  GraphicEmissiveColor=[clr_emblem_f 1.0]  GraphicShininess=75  DoExposeReferenceFrame=on  SerializedFrames=<Frames/>
  Ornament Rear : sm_lib/Body Elements/Extruded Solid  ExtrusionType=General  PolygonNumSides=3  PolygonOuterRadius=1  PolygonOuterRadiusUnits=m  ExportEntireGeometry=off  ExtrusionCrossSection=extr_data_emblem_r  ExtrusionCrossSectionUnits=m  ExportConvexHullGeometry=off  ExtrusionLength=0.01  ExtrusionLengthUnits=m  InertiaType=CalculateFromGeometry  BasedOnType=Density  Density=1000  DensityUnits=kg/m^3  Mass=1  MassUnits=kg  CenterOfMass=[0 0 0]  CenterOfMassUnits=m  MomentsOfInertia=[1 1 1]  MomentsOfInertiaUnits=kg*m^2  ProductsOfInertia=[0 0 0]  ProductsOfInertiaUnits=kg*m^2  GraphicType=FromGeometry  MarkerShape=Sphere  MarkerSize=10  GraphicVisPropType=SimpleVisualProperties  GraphicDiffuseColor=clr_emblem_r  GraphicOpacity=opc_emblem_r  GraphicSpecularColor=[0.5 0.5 0.5 1.0]  GraphicAmbientColor=[0.15 0.15 0.15 1.0]  GraphicEmissiveColor=[0.0 0.0 0.0 1.0]  GraphicShininess=75  DoExposeReferenceFrame=on  SerializedFrames=<Frames/>
  Rear View : sm_lib/Frames and Transforms/Reference Frame
  Right Face : sm_lib/Body Elements/Extruded Solid  ExtrusionType=General  PolygonNumSides=3  PolygonOuterRadius=1  PolygonOuterRadiusUnits=m  ExportEntireGeometry=off  ExtrusionCrossSection=xy_data_car_side  ExtrusionCrossSectionUnits=m  ExportConvexHullGeometry=off  ExtrusionLength=thk_side  ExtrusionLengthUnits=m  InertiaType=PointMass  BasedOnType=Density  Density=1000  DensityUnits=kg/m^3  Mass=0  MassUnits=kg  CenterOfMass=[0 0 0]  CenterOfMassUnits=m  MomentsOfInertia=[1 1 1]  MomentsOfInertiaUnits=kg*m^2  ProductsOfInertia=[0 0 0]  ProductsOfInertiaUnits=kg*m^2  GraphicType=FromGeometry  MarkerShape=Sphere  MarkerSize=10  GraphicVisPropType=SimpleVisualProperties  GraphicDiffuseColor=clr_body_geo_right  GraphicOpacity=opc_body_geo_right  GraphicSpecularColor=[0.5 0.5 0.5 1.0]  GraphicAmbientColor=[0.15 0.15 0.15 1.0]  GraphicEmissiveColor=[0.0 0.0 0.0 1.0]  GraphicShininess=75  DoExposeReferenceFrame=on  SerializedFrames=<Frames/>
  Top Surface : sm_lib/Body Elements/Extruded Solid  ExtrusionType=General  PolygonNumSides=3  PolygonOuterRadius=1  PolygonOuterRadiusUnits=m  ExportEntireGeometry=off  ExtrusionCrossSection=xy_data_car_top  ExtrusionCrossSectionUnits=m  ExportConvexHullGeometry=off  ExtrusionLength=car_track  ExtrusionLengthUnits=m  InertiaType=PointMass  BasedOnType=Density  Density=0  DensityUnits=kg/m^3  Mass=0  MassUnits=kg  CenterOfMass=[0 0 0]  CenterOfMassUnits=m  MomentsOfInertia=[1 1 1]  MomentsOfInertiaUnits=kg*m^2  ProductsOfInertia=[0 0 0]  ProductsOfInertiaUnits=kg*m^2  GraphicType=FromGeometry  MarkerShape=Sphere  MarkerSize=10  GraphicVisPropType=SimpleVisualProperties  GraphicDiffuseColor=clr_body_geo_top  GraphicOpacity=opc_body_geo_top  GraphicSpecularColor=[0.5 0.5 0.5 1.0]  GraphicAmbientColor=[0.15 0.15 0.15 1.0]  GraphicEmissiveColor=[0.0 0.0 0.0 1.0]  GraphicShininess=75  DoExposeReferenceFrame=on  SerializedFrames=<Frames/>
  Transform Extrusion Axes : sm_lib/Frames and Transforms/Rigid Transform  RotationMethod=StandardAxis  FollAlignAxisA=+X  BaseAlignAxisA=+Y  FollAlignAxisB=+Y  BaseAlignAxisB=+Z  RotationStandardAxis=+X  RotationAngle=90  RotationAngleUnits=deg  RotationArbitraryAxis=[0 0 1]  RotationSequenceAxes=FollowerAxes  RotationSequence=XYX  RotationSequenceAngles=[0 0 0]  RotationSequenceAnglesUnits=deg  RotationMatrix=[1 0 0; 0 1 0; 0 0 1]  Quaternion=[1 0 0 0]  TranslationMethod=None  TranslationCartesianOffset=[0 0 0]  TranslationCartesianOffsetUnits=m  TranslationStandardAxis=+Z  TranslationStandardOffset=0  TranslationStandardOffsetUnits=m  TranslationROffset=0  TranslationROffsetUnits=m  TranslationThetaOffset=0  TranslationThetaOffsetUnits=deg  TranslationZOffset=0  TranslationZOffsetUnits=m
  Transform Ornament Front : sm_lib/Frames and Transforms/Rigid Transform  RotationMethod=RotationSequence  FollAlignAxisA=+X  BaseAlignAxisA=+Y  FollAlignAxisB=+Y  BaseAlignAxisB=+Z  RotationStandardAxis=+Z  RotationAngle=90  RotationAngleUnits=deg  RotationArbitraryAxis=[0 0 1]  RotationSequenceAxes=FollowerAxes  RotationSequence=ZXY  RotationSequenceAngles=[90 90 0]  RotationSequenceAnglesUnits=deg  RotationMatrix=[1 0 0; 0 1 0; 0 0 1]  Quaternion=[1 0 0 0]  TranslationMethod=Cartesian  TranslationCartesianOffset=[max(xy_data_car_side(:,1)) 0 min(xy_data_car_side(:,2))+0.15]  TranslationCartesianOffsetUnits=m  TranslationStandardAxis=+Z  TranslationStandardOffset=1  TranslationStandardOffsetUnits=m  TranslationROffset=0  TranslationROffsetUnits=m  TranslationThetaOffset=0  TranslationThetaOffsetUnits=deg  TranslationZOffset=0  TranslationZOffsetUnits=m
  Transform Ornament Rear : sm_lib/Frames and Transforms/Rigid Transform  RotationMethod=RotationSequence  FollAlignAxisA=+X  BaseAlignAxisA=+Y  FollAlignAxisB=+Y  BaseAlignAxisB=+Z  RotationStandardAxis=+Z  RotationAngle=90  RotationAngleUnits=deg  RotationArbitraryAxis=[0 0 1]  RotationSequenceAxes=FollowerAxes  RotationSequence=ZXY  RotationSequenceAngles=[90 90 180]  RotationSequenceAnglesUnits=deg  RotationMatrix=[1 0 0; 0 1 0; 0 0 1]  Quaternion=[1 0 0 0]  TranslationMethod=Cartesian  TranslationCartesianOffset=[min(xy_data_car_side(:,1))+0.1 0 min(xy_data_car_side(:,2))+0.15]  TranslationCartesianOffsetUnits=m  TranslationStandardAxis=+Z  TranslationStandardOffset=1  TranslationStandardOffsetUnits=m  TranslationROffset=0  TranslationROffsetUnits=m  TranslationThetaOffset=0  TranslationThetaOffsetUnits=deg  TranslationZOffset=0  TranslationZOffsetUnits=m
  Transform Rear View : sm_lib/Frames and Transforms/Rigid Transform  RotationMethod=None  FollAlignAxisA=+X  BaseAlignAxisA=+Y  FollAlignAxisB=+Y  BaseAlignAxisB=+Z  RotationStandardAxis=+Z  RotationAngle=0.0  RotationAngleUnits=deg  RotationArbitraryAxis=[0 0 1]  RotationSequenceAxes=FollowerAxes  RotationSequence=XYX  RotationSequenceAngles=[0 0 0]  RotationSequenceAnglesUnits=deg  RotationMatrix=[1 0 0; 0 1 0; 0 0 1]  Quaternion=[1 0 0 0]  TranslationMethod=Cartesian  TranslationCartesianOffset=[min(xy_data_car_side(:,1))-4 0 min(xy_data_car_side(:,2))+1]  TranslationCartesianOffsetUnits=m  TranslationStandardAxis=+Z  TranslationStandardOffset=0  TranslationStandardOffsetUnits=m  TranslationROffset=0  TranslationROffsetUnits=m  TranslationThetaOffset=0  TranslationThetaOffsetUnits=deg  TranslationZOffset=0  TranslationZOffsetUnits=m
  Transform Reference : sm_lib/Frames and Transforms/Rigid Transform  RotationMethod=None  FollAlignAxisA=+X  BaseAlignAxisA=+Y  FollAlignAxisB=+Y  BaseAlignAxisB=+Z  RotationStandardAxis=+Z  RotationAngle=0.0  RotationAngleUnits=deg  RotationArbitraryAxis=[0 0 1]  RotationSequenceAxes=FollowerAxes  RotationSequence=XYX  RotationSequenceAngles=[0 0 0]  RotationSequenceAnglesUnits=deg  RotationMatrix=[1 0 0; 0 1 0; 0 0 1]  Quaternion=[1 0 0 0]  TranslationMethod=Cartesian  TranslationCartesianOffset=offset_ref  TranslationCartesianOffsetUnits=m  TranslationStandardAxis=+Z  TranslationStandardOffset=0  TranslationStandardOffsetUnits=m  TranslationROffset=0  TranslationROffsetUnits=m  TranslationThetaOffset=0  TranslationThetaOffsetUnits=deg  TranslationZOffset=0  TranslationZOffsetUnits=m
  Transform Left Face : sm_lib/Frames and Transforms/Rigid Transform  RotationMethod=None  FollAlignAxisA=+X  BaseAlignAxisA=+Y  FollAlignAxisB=+Y  BaseAlignAxisB=+Z  RotationStandardAxis=+Z  RotationAngle=0.0  RotationAngleUnits=deg  RotationArbitraryAxis=[0 0 1]  RotationSequenceAxes=FollowerAxes  RotationSequence=XYX  RotationSequenceAngles=[0 0 0]  RotationSequenceAnglesUnits=deg  RotationMatrix=[1 0 0; 0 1 0; 0 0 1]  Quaternion=[1 0 0 0]  TranslationMethod=StandardAxis  TranslationCartesianOffset=[0 0 0]  TranslationCartesianOffsetUnits=m  TranslationStandardAxis=-Z  TranslationStandardOffset=car_track/2-thk_side/2  TranslationStandardOffsetUnits=m  TranslationROffset=0  TranslationROffsetUnits=m  TranslationThetaOffset=0  TranslationThetaOffsetUnits=deg  TranslationZOffset=0  TranslationZOffsetUnits=m
  Transform Right Face : sm_lib/Frames and Transforms/Rigid Transform  RotationMethod=None  FollAlignAxisA=+X  BaseAlignAxisA=+Y  FollAlignAxisB=+Y  BaseAlignAxisB=+Z  RotationStandardAxis=+Z  RotationAngle=0.0  RotationAngleUnits=deg  RotationArbitraryAxis=[0 0 1]  RotationSequenceAxes=FollowerAxes  RotationSequence=XYX  RotationSequenceAngles=[0 0 0]  RotationSequenceAnglesUnits=deg  RotationMatrix=[1 0 0; 0 1 0; 0 0 1]  Quaternion=[1 0 0 0]  TranslationMethod=StandardAxis  TranslationCartesianOffset=[0 0 0]  TranslationCartesianOffsetUnits=m  TranslationStandardAxis=+Z  TranslationStandardOffset=car_track/2-thk_side/2  TranslationStandardOffsetUnits=m  TranslationROffset=0  TranslationROffsetUnits=m  TranslationThetaOffset=0  TranslationThetaOffsetUnits=deg  TranslationZOffset=0  TranslationZOffsetUnits=m
  FA : PMIOPort  Side=Right
  P : PMIOPort  Port=2  Side=Left
  connections:
  Transform Reference/LConn1 -- P/RConn1 -- FA/RConn1
  Transform Rear View/RConn1 -- Rear View/RConn1
  Transform Reference/RConn1 -- Transform Ornament Front/LConn1 -- Transform Ornament Rear/LConn1 -- Transform Rear View/LConn1 -- Transform Extrusion Axes/LConn1
  Left Face/RConn1 -- Transform Left Face/RConn1
  Transform Extrusion Axes/RConn1 -- Transform Right Face/LConn1 -- Top Surface/RConn1 -- Transform Left Face/LConn1
  Right Face/RConn1 -- Transform Right Face/RConn1
  Transform Ornament Front/RConn1 -- Ornament Front/RConn1
  Transform Ornament Rear/RConn1 -- Ornament Rear/RConn1

== system sm_car/Vehicle/Vehicle/Body to World/Free/R to X-Y-Z Extrinsic ==
  note: The sensor implemented here computes roll / pitch / yaw values assuming they correpsond to X, Y, and Z rotations, applied in that order and using  *extrinsic* rotations.  That is, the rotations are applied about the fixed (non-rotated) axes of the base frame.   There are many other possible conventions, but the computations of angles has the same basic structure for any of them.  The only differences would be which elements of the rotation matrix are picked off for analysis, and which signals are negated.
      |
      | This implementation does not handle the gimbal-lock case robustly, which occurs when the Y (pitch) rotation is +/-90 degrees.  Handling this case requires a more complex computation,
      | but it can be done with a few more trig blocks and selectors.
  R : Inport
  Asin : Trigonometry  Operator=asin
  Atan1 : Trigonometry  Operator=atan2
  Atan2 : Trigonometry  Operator=atan2
  Demux : Demux  Outputs=2
  Demux1 : Demux  Outputs=2
  Multiply2 : Gain  Gain=-1
  "R(3, 1)" : Selector  NumberOfDimensions=2  InputPortWidth=3  IndexOptions=Index vector (dialog),Index vector (dialog)  Indices=3,1  OutputSizes=1,1
  "R(3, 2:3)" : Selector  NumberOfDimensions=2  InputPortWidth=3  IndexOptions=Index vector (dialog),Index vector (dialog)  Indices=3,[2 3]  OutputSizes=1,1
  "R([2 1], 1)" : Selector  NumberOfDimensions=2  InputPortWidth=3  IndexOptions=Index vector (dialog),Index vector (dialog)  Indices=[2 1],1  OutputSizes=1,1
  Reshape : Reshape
  Reshape1 : Reshape
  Reshape2 : Reshape  OutputDimensionality=Customize  OutputDimensions=1
  yaw : Outport  VectorParamsAs1DForOutWhenUnconnected=off
  pitch : Outport  Port=2  VectorParamsAs1DForOutWhenUnconnected=off
  roll : Outport  Port=3  VectorParamsAs1DForOutWhenUnconnected=off
  wires:
  Reshape2/1 -> roll/1
  Reshape1/1 -> pitch/1
  Reshape/1 -> yaw/1
  Atan1/1 -> Reshape/1
  "R(3, 2:3)"/1 -> Demux/1
  Multiply2/1 -> Asin/1
  "R([2 1], 1)"/1 -> Demux1/1
  Demux1/1 -> Atan1/1
  R/1 -> "R([2 1], 1)"/1, "R(3, 2:3)"/1, "R(3, 1)"/1
  Asin/1 -> Reshape1/1
  "R(3, 1)"/1 -> Multiply2/1
  Atan2/1 -> Reshape2/1
  Demux/2 -> Atan2/2
  Demux1/2 -> Atan1/2
  Demux/1 -> Atan2/1

== system sm_car/Vehicle/Vehicle/Brakes/PedalAbstract DiscDisc/Actuator L1 ==
  Pedal : Inport
  Filter : TransferFcn  Numerator=brk_max_p  Denominator=[brk_filt 1]
  Simulink-PS Converter : nesl_utility/Simulink-PS Converter  PhysicalDomain=network_engine_domain  SubClassName=ps_input  LeftPortType=input  RightPortType=output  PseudoPeriodic=off  Frequencies=[]  NoiseDistribution=none  NoiseParameters=[]  Unit=1  AffineConversion=off  FilteringAndDerivatives=provide  SimscapeFilterOrder=1  InputFilterTimeConstant=0.001  UdotUserProvided=0
  P : PMIOPort  Side=Right
  wires:
  Pedal/1 -> Filter/1
  Filter/1 -> Simulink-PS Converter/1
  connections:
  Simulink-PS Converter/RConn1 -- P/RConn1

== system sm_car/Vehicle/Vehicle/Brakes/PedalAbstract DiscDisc/Actuator L2 ==
  Pedal : Inport
  Filter : TransferFcn  Numerator=brk_max_p  Denominator=[brk_filt 1]
  Simulink-PS Converter : nesl_utility/Simulink-PS Converter  PhysicalDomain=network_engine_domain  SubClassName=ps_input  LeftPortType=input  RightPortType=output  PseudoPeriodic=off  Frequencies=[]  NoiseDistribution=none  NoiseParameters=[]  Unit=1  AffineConversion=off  FilteringAndDerivatives=provide  SimscapeFilterOrder=1  InputFilterTimeConstant=0.001  UdotUserProvided=0
  P : PMIOPort  Side=Right
  wires:
  Pedal/1 -> Filter/1
  Filter/1 -> Simulink-PS Converter/1
  connections:
  Simulink-PS Converter/RConn1 -- P/RConn1

== system sm_car/Vehicle/Vehicle/Brakes/PedalAbstract DiscDisc/Actuator R1 ==
  Pedal : Inport
  Filter : TransferFcn  Numerator=brk_max_p  Denominator=[brk_filt 1]
  Simulink-PS Converter : nesl_utility/Simulink-PS Converter  PhysicalDomain=network_engine_domain  SubClassName=ps_input  LeftPortType=input  RightPortType=output  PseudoPeriodic=off  Frequencies=[]  NoiseDistribution=none  NoiseParameters=[]  Unit=1  AffineConversion=off  FilteringAndDerivatives=provide  SimscapeFilterOrder=1  InputFilterTimeConstant=0.001  UdotUserProvided=0
  P : PMIOPort  Side=Right
  wires:
  Pedal/1 -> Filter/1
  Filter/1 -> Simulink-PS Converter/1
  connections:
  Simulink-PS Converter/RConn1 -- P/RConn1

== system sm_car/Vehicle/Vehicle/Brakes/PedalAbstract DiscDisc/Actuator R2 ==
  Pedal : Inport
  Filter : TransferFcn  Numerator=brk_max_p  Denominator=[brk_filt 1]
  Simulink-PS Converter : nesl_utility/Simulink-PS Converter  PhysicalDomain=network_engine_domain  SubClassName=ps_input  LeftPortType=input  RightPortType=output  PseudoPeriodic=off  Frequencies=[]  NoiseDistribution=none  NoiseParameters=[]  Unit=1  AffineConversion=off  FilteringAndDerivatives=provide  SimscapeFilterOrder=1  InputFilterTimeConstant=0.001  UdotUserProvided=0
  P : PMIOPort  Side=Right
  wires:
  Pedal/1 -> Filter/1
  Filter/1 -> Simulink-PS Converter/1
  connections:
  Simulink-PS Converter/RConn1 -- P/RConn1

== system sm_car/Vehicle/Vehicle/Brakes/PedalAbstract DiscDisc/Sensing Torque L1 ==
  Ideal Torque Sensor : fl_lib/Mechanical/Mechanical Sensors/Ideal Torque Sensor
  PS-Simulink Converter : nesl_utility/PS-Simulink Converter  PhysicalDomain=network_engine_domain  SubClassName=ps_output  LeftPortType=input  RightPortType=output  PseudoPeriodic=off  Frequencies=[]  VectorFormat=1-D array  Unit=N*m  AffineConversion=off
  C : PMIOPort  Side=Right
  R : PMIOPort  Port=2  Side=Left
  T : Outport  VectorParamsAs1DForOutWhenUnconnected=off
  wires:
  PS-Simulink Converter/1 -> T/1
  connections:
  PS-Simulink Converter/LConn1 -- Ideal Torque Sensor/RConn2
  Ideal Torque Sensor/RConn1 -- C/RConn1
  Ideal Torque Sensor/LConn1 -- R/RConn1

== system sm_car/Vehicle/Vehicle/Brakes/PedalAbstract DiscDisc/Sensing Torque L2 ==
  Ideal Torque Sensor : fl_lib/Mechanical/Mechanical Sensors/Ideal Torque Sensor
  PS-Simulink Converter : nesl_utility/PS-Simulink Converter  PhysicalDomain=network_engine_domain  SubClassName=ps_output  LeftPortType=input  RightPortType=output  PseudoPeriodic=off  Frequencies=[]  VectorFormat=1-D array  Unit=N*m  AffineConversion=off
  C : PMIOPort  Side=Right
  R : PMIOPort  Port=2  Side=Left
  T : Outport  VectorParamsAs1DForOutWhenUnconnected=off
  wires:
  PS-Simulink Converter/1 -> T/1
  connections:
  PS-Simulink Converter/LConn1 -- Ideal Torque Sensor/RConn2
  Ideal Torque Sensor/RConn1 -- C/RConn1
  Ideal Torque Sensor/LConn1 -- R/RConn1

== system sm_car/Vehicle/Vehicle/Brakes/PedalAbstract DiscDisc/Sensing Torque R1 ==
  Ideal Torque Sensor : fl_lib/Mechanical/Mechanical Sensors/Ideal Torque Sensor
  PS-Simulink Converter : nesl_utility/PS-Simulink Converter  PhysicalDomain=network_engine_domain  SubClassName=ps_output  LeftPortType=input  RightPortType=output  PseudoPeriodic=off  Frequencies=[]  VectorFormat=1-D array  Unit=N*m  AffineConversion=off
  C : PMIOPort  Side=Right
  R : PMIOPort  Port=2  Side=Left
  T : Outport  VectorParamsAs1DForOutWhenUnconnected=off
  wires:
  PS-Simulink Converter/1 -> T/1
  connections:
  Ideal Torque Sensor/LConn1 -- R/RConn1
  Ideal Torque Sensor/RConn1 -- C/RConn1
  PS-Simulink Converter/LConn1 -- Ideal Torque Sensor/RConn2

== system sm_car/Vehicle/Vehicle/Brakes/PedalAbstract DiscDisc/Sensing Torque R2 ==
  Ideal Torque Sensor : fl_lib/Mechanical/Mechanical Sensors/Ideal Torque Sensor
  PS-Simulink Converter : nesl_utility/PS-Simulink Converter  PhysicalDomain=network_engine_domain  SubClassName=ps_output  LeftPortType=input  RightPortType=output  PseudoPeriodic=off  Frequencies=[]  VectorFormat=1-D array  Unit=N*m  AffineConversion=off
  C : PMIOPort  Side=Right
  R : PMIOPort  Port=2  Side=Left
  T : Outport  VectorParamsAs1DForOutWhenUnconnected=off
  wires:
  PS-Simulink Converter/1 -> T/1
  connections:
  Ideal Torque Sensor/LConn1 -- R/RConn1
  Ideal Torque Sensor/RConn1 -- C/RConn1
  PS-Simulink Converter/LConn1 -- Ideal Torque Sensor/RConn2
